simulink library "Steer_Rack_None"  (R2025a)
settings: Solver=VariableStepAuto  StartTime=0.0  StopTime=10.0  RelTol=1e-3
libraries: Body_Utilities x1, Vehicle_Inputs x1
Description:
  | Component of Simscape Vehicle Templates Library
  | 
  | Copyright 2018-2026 The MathWorks, Inc.
settings Model: Creator=smiller  LastModifiedBy=smiller
settings OptimizationCC: ReuseModelBlockBuffer=off
settings ModelReferenceCC: EnableRefExpFcnMdlSchedulingChecks=on
settings RTWCC: GPUComputeCapability=3.5

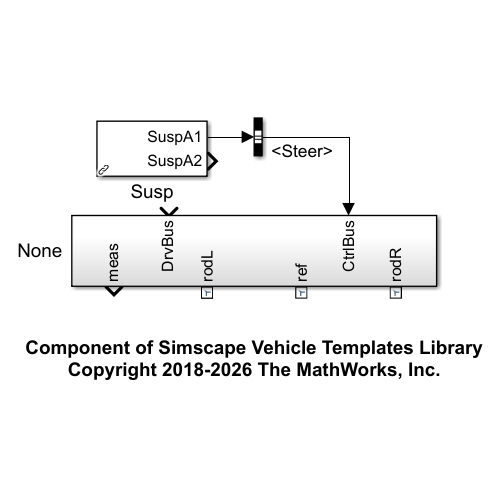
[thumbnail: Simulink's stored preview of the top-level diagram]
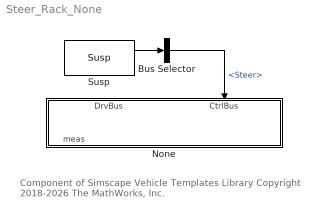
== system Steer_Rack_None ==
  note: Component of Simscape Vehicle Templates Library
      | Copyright 2018-2026 The MathWorks, Inc.
  Bus Selector : BusSelector  OutputSignals=Steer
  None : Subsystem  VariantControl=None
  Susp : Vehicle_Inputs/Control Bus/Susp  SystemSampleTime=-1  VariantActivationTime=update diagram  EmptyChoice=off  PassThrough=off  PassThroughVariantControl=(default)  EmptyChoiceVariantControl=(default)  AllowFlexibleInterface=on  Latency=0  AutoFrameSizeCalculation=off
  wires:
  Bus Selector/1 -> None/2(CtrlBus)  "<Steer>"
  Susp/1 -> Bus Selector/1

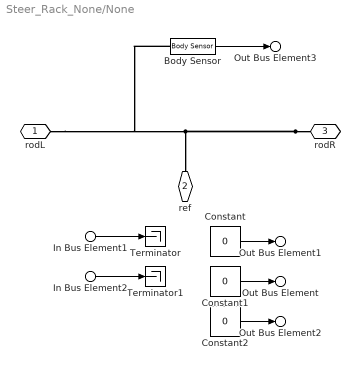
== system Steer_Rack_None/None ==
  In Bus Element1 : Inport  PortName=DrvBus  Element=aSteerWheel
  In Bus Element2 : Inport  Port=2  PortName=CtrlBus
  Body Sensor : Body_Utilities/Body Sensor  offset_body_sensor=Vehicle.Chassis.Body.sCG.Value
  Constant : Constant  Value=0
  Constant1 : Constant  Value=0
  Constant2 : Constant  Value=0
  Terminator : Terminator
  Terminator1 : Terminator
  rodL : PMIOPort  Side=Right
  ref : PMIOPort  Port=2  Side=Right
  rodR : PMIOPort  Port=3  Side=Right
  Out Bus Element : Outport  VectorParamsAs1DForOutWhenUnconnected=off  PortName=meas  Element=FRack
  Out Bus Element1 : Outport  VectorParamsAs1DForOutWhenUnconnected=off  PortName=meas  Element=xRack
  Out Bus Element2 : Outport  VectorParamsAs1DForOutWhenUnconnected=off  PortName=meas  Element=aWheel
  Out Bus Element3 : Outport  VectorParamsAs1DForOutWhenUnconnected=off  PortName=meas  Element=Driver
  wires:
  Body Sensor/1 -> Out Bus Element3/1
  Constant2/1 -> Out Bus Element2/1
  In Bus Element2/1 -> Terminator1/1
  Constant1/1 -> Out Bus Element/1
  Constant/1 -> Out Bus Element1/1
  In Bus Element1/1 -> Terminator/1
  connections:
  rodR/RConn1 -- ref/RConn1 -- Body Sensor/LConn1 -- rodL/RConn1
